simulink model "W10_PID_AntiWindup"  (R2024b)
settings: Solver=ode45  StartTime=0.0  StopTime=t_end  MaxStep=0.002  RelTol=1e-3
PreLoadFcn:
  | % W10_PID_AntiWindup 기본 파라미터 (모델을 열 때 자동 실행)
  | % 플랜트는 DC 모터 속도 모델 (CTMS 표준값)
  | defs = { 'Kp',60 ; 'Ki',400 ; 'Kd',0 ; 'Nf',100 ;
  |          'r_amp',1 ; 'u_max',15 ; 't_end',2.5 ;
  |          'Kb_gain',1 ;
  |          'numG',0.01 ; 'denG',[0.005 0.06 0.1001] };
  | for ii = 1:size(defs,1)
  |     if ~evalin('base', sprintf('exist(''%s'',''var'')', defs{ii,1}))
  |         assignin('base', defs{ii,1}, defs{ii,2});
  |     end
  | end
  | clear defs ii
values from neighbouring files (symbols this model uses):
  Kb_gain = 20    [W10_04_run_simulink.m]
  Kd = 10    [W10_03_pid_tuning.m]    (also in W10_04_run_simulink.m = 0)
  Ki = 200    [W10_03_pid_tuning.m]    (also in W10_04_run_simulink.m = 400)
  Kp = 100    [W10_03_pid_tuning.m]    (also in W10_04_run_simulink.m = 60)
  Nf = 100    [W10_03_pid_tuning.m]    (also in W10_04_run_simulink.m)
  r_amp = 1    [W10_04_run_simulink.m]
  u_max = 15    [W10_04_run_simulink.m]
undefined symbols (not defined in the file or in its folder): denG, numG
libraries: slpidlib x1
settings Model: Creator=admin  LastModifiedBy=admin
settings SolverCC: ZeroCrossAlgorithm=Adaptive
settings DebuggingCC: IgnoredZcDiagnostic=none

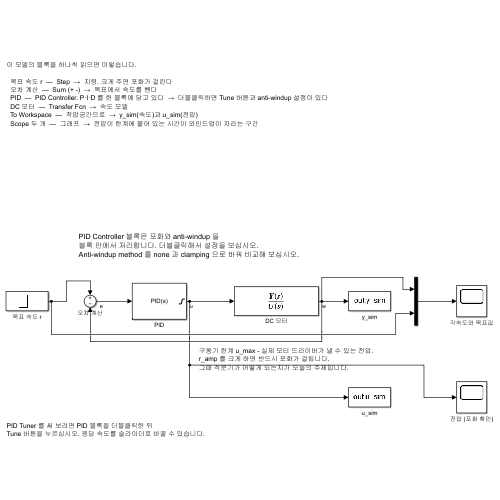
[thumbnail: Simulink's stored preview of the top-level diagram]
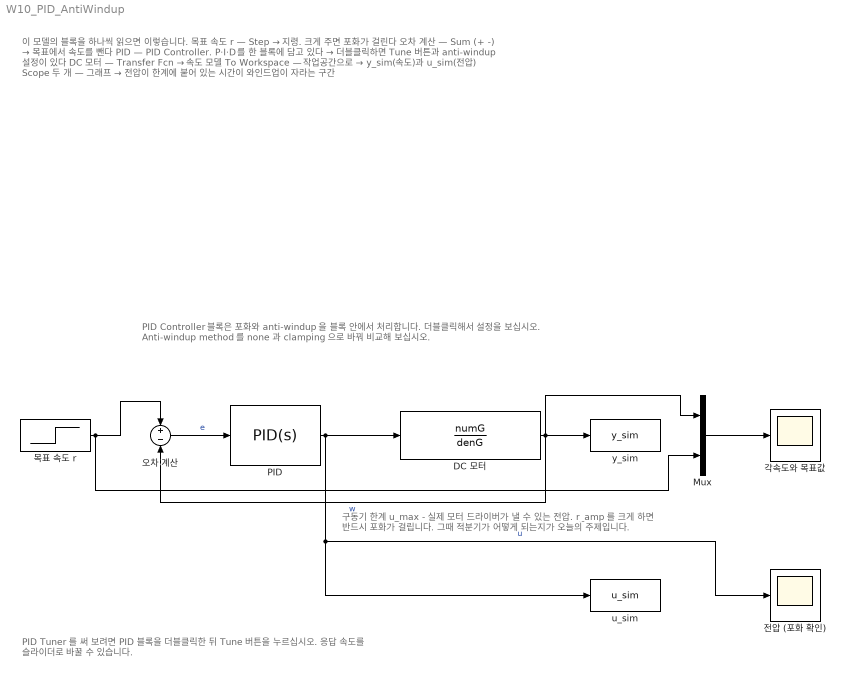
== system W10_PID_AntiWindup ==
  note: PID Controller 블록은 포화와 anti-windup 을
      | 블록 안에서 처리합니다. 더블클릭해서 설정을 보십시오.
      | Anti-windup method 를 none 과 clamping 으로 바꿔 비교해 보십시오.
  note: 구동기 한계 u_max - 실제 모터 드라이버가 낼 수 있는 전압.
      | r_amp 를 크게 하면 반드시 포화가 걸립니다.
      | 그때 적분기가 어떻게 되는지가 오늘의 주제입니다.
  note: PID Tuner 를 써 보려면 PID 블록을 더블클릭한 뒤
      | Tune 버튼을 누르십시오. 응답 속도를 슬라이더로 바꿀 수 있습니다.
  note: 이 모델의 블록을 하나씩 읽으면 이렇습니다.
      |
      |   목표 속도 r  —  Step  →  지령. 크게 주면 포화가 걸린다
      |   오차 계산  —  Sum (+ -)  →  목표에서 속도를 뺀다
      |   PID  —  PID Controller. P·I·D 를 한 블록에 담고 있다  →  더블클릭하면 Tune 버튼과 anti-windup 설정이 있다
      |   DC 모터  —  Transfer Fcn  →  속도 모델
      |   To Workspace  —  작업공간으로  →  y_sim(속도)과 u_sim(전압)
      |   Scope 두 개  —  그래프  →  전압이 한계에 붙어 있는 시간이 와인드업이 자라는 구간
  DC 모터 : TransferFcn  Numerator=numG  Denominator=denG
  Mux : Mux  Inputs=2
  PID : slpidlib/PID Controller  Controller=PID  Form=Parallel  TimeDomain=Continuous-time  UseExternalTs=off  SampleTime=-1  IntegratorMethod=Forward Euler  FilterMethod=Forward Euler  ControllerParametersSource=internal  P=Kp  I=Ki  UseKiTs=off  D=Kd  UseExternalDerivativeSource=off  N=Nf  UseFilter=on  TunerSelectOption=Transfer Function Based (PID Tuner App)  InitialConditionSource=internal  InitialConditionForIntegrator=0  InitialConditionForFilter=0  DifferentiatorICPrevScaledInput=0  ExternalReset=none  TrackingMode=off  Kt=1  LimitOutput=on  SatLimitsSource=internal  UpperSaturationLimit=u_max  LowerSaturationLimit=-u_max  LinearizeAsGain=on  AntiWindupMode=none  Kb=Kb_gain  LimitIntegrator=off  UpperIntegratorSaturationLimit=inf  LowerIntegratorSaturationLimit=-inf  POutMin=[]  POutMax=[]  IOutMin=[]  IOutMax=[]  DOutMin=[]  DOutMax=[]  NOutMin=[]  NOutMax=[]  SumOutMin=[]  SumOutMax=[]  SaturationOutMin=[]  SaturationOutMax=[]  PParamMin=[]  PParamMax=[]  IParamMin=[]  IParamMax=[]  DParamMin=[]  DParamMax=[]  NParamMin=[]  NParamMax=[]  KbParamMin=[]  KbParamMax=[]  KtParamMin=[]  KtParamMax=[]  KbOutMin=[]  KbOutMax=[]  KtOutMin=[]  KtOutMax=[]  IntegratorOutMin=[]  IntegratorOutMax=[]  FilterOutMin=[]  FilterOutMax=[]  SumI1OutMin=[]  SumI1OutMax=[]  SumI2OutMin=[]  SumI2OutMax=[]  SumI3OutMin=[]  SumI3OutMax=[]  SumI4OutMin=[]  SumI4OutMax=[]  SumDOutMin=[]  SumDOutMax=[]  DifferentiatorOutMin=[]  DifferentiatorOutMax=[]  FilterDiffOutCoefMin=[]  FilterDiffOutCoefMax=[]  ReciprocalOutMin=[]  ReciprocalOutMax=[]  SumDenOutMin=[]  SumDenOutMax=[]  SumNumOutMin=[]  SumNumOutMax=[]  DivideOutMin=[]  DivideOutMax=[]  UdiffTsProdOutMin=[]  UdiffTsProdOutMax=[]  NTsProdOutMin=[]  NTsProdOutMax=[]  UintegralTsProdOutMin=[]  UintegralTsProdOutMax=[]  UngainTsProdOutMin=[]  UngainTsProdOutMax=[]  ClampingZeroOutDataTypeStr=Inherit: Inherit via back propagation  ClampingZeroOutMin=[]  ClampingZeroOutMax=[]  FilterDenConstantOutDataTypeStr=Inherit: Inherit via back propagation  FilterDenConstantOutMin=[]  FilterDenConstantOutMax=[]  PCopyOutDataTypeStr=Inherit: Inherit via back propagation  PCopyOutMin=[]  PCopyOutMax=[]  NCopyOutDataTypeStr=Inherit: Inherit via back propagation  NCopyOutMin=[]  NCopyOutMax=[]  IntegratorContinuousStateAttributes=''  IntegratorStateMustResolveToSignalObject=off  IntegratorRTWStateStorageClass=Auto  FilterContinuousStateAttributes=''  FilterStateMustResolveToSignalObject=off  FilterRTWStateStorageClass=Auto  ParallelPVariant=InternalParameters  IdealPVariant=Disabled  IVariant=InternalParameters  DVariant=InternalParameters  IntegratorVariant=Continuous  SatVariant=Enabled  AWVariant=Passthrough  PCopyVariant=Disabled  TRVariant=Disabled  FdbkBlocksVariant=Forward  IdealPFdbkVariant=Disabled  SatFdbkVariant=Disabled  DerivativeFilterVariant=ContFilter  NVariant=InternalParameters  NCopyVariant=Disabled  FilterICVariant=InternalICsFilter  IntegratorICVariant=InternalICs  ExternalResetVariant=Disabled  TRSumVariant=Passthrough  SumFdbkVariant=Disabled  SumVariant=Sum_PID  TsampFilterVariant=InternalTs  TsampNgainVariant=Passthrough  TsampIntegralVariant=Disabled_SignalSpec  ExternalSaturationOutDataTypeStr=Inherit: Same as second input  DerivativeSourceVariant=ErrorSignal  PreIntVariant=InternalPreInt
  u_sim : ToWorkspace  VariableName=u_sim  SaveFormat=Timeseries  SampleTime=-1
  y_sim : ToWorkspace  VariableName=y_sim  SaveFormat=Timeseries  SampleTime=-1
  각속도와 목표값 : Scope
  목표 속도 r : Step  Time=0  After=r_amp  SampleTime=0
  오차 계산 : Sum  Inputs=+-
  전압 (포화 확인) : Scope
  wires:
  목표 속도 r/1 -> 오차 계산/1, Mux/2
  오차 계산/1 -> PID/1  "e"
  PID/1 -> u_sim/1, 전압 (포화 확인)/1, DC 모터/1  "u"
  DC 모터/1 -> y_sim/1, 오차 계산/2, Mux/1  "w"
  Mux/1 -> 각속도와 목표값/1
